simulink model "heatdrive_ecc_coupled_se21"  (R2025b)
settings: Solver=ode23t  StartTime=0.0  StopTime=10  FixedStep=0.1  MaxStep=0.4  RelTol=1e-2  AbsTol=1e-3
values from neighbouring files (symbols this model uses):
  cold_load_heat_W = 0.0    (= 0)    [Build_Simulink_Exchange_Params.m]
  cold_load_T_init = get_stage_field(stage_config, 'cold_load_T_in', get_stage_field(stage_config,          'chip_T_in', get_option_field(exchange_options, 'cold_load_T_init', get_option_field(exchange_options, 'chip_T_init', 293.0))))    [Build_Simulink_Exchange_Params.m]    (also in Create_Simulink_Exchange_Runtime.m = get_option_field(options, 'cold_load_T_init',          get_o)
  cold_sink_T_init = get_stage_field(stage_config, 'cold_sink_T_in', get_option_field(exchange_options, 'cold_sink_T_init', 293.0))    [Build_Simulink_Exchange_Params.m]    (also in Create_Simulink_Exchange_Runtime.m = get_option_field(options, 'cold_sink_T_init', ambient_T_init)
  hot_sink_T_init = get_stage_field(stage_config, 'hot_sink_T_in', get_option_field(exchange_options, 'hot_sink_T_init', 293.0))    [Build_Simulink_Exchange_Params.m]    (also in Create_Simulink_Exchange_Runtime.m = get_option_field(options, 'hot_sink_T_init', ambient_T_init))
  mdot_cooldown_source_kgps = mdot_target_kgps    [Build_Simulink_Exchange_Params.m]
  mdot_hold_source_kgps = mdot_target_kgps    [Build_Simulink_Exchange_Params.m]
  pressure_pi_bias_MPa = pressure_pi_dp_guess_MPa    [Build_Simulink_Exchange_Params.m]
  pressure_pi_error_filter_tau_s = max(get_option_field(exchange_options, 'pressure_pi_error_filter_tau_s', 0.002), 1.0e-5)    [Build_Simulink_Exchange_Params.m]
  pressure_pi_error_normalization_gain_kgps_inv = 1.0    (= 1)    [Build_Simulink_Exchange_Params.m]
  pressure_pi_max_MPa = pressure_pi_dp_guess_MPa + pressure_pi_margin_MPa    [Build_Simulink_Exchange_Params.m]
  shex_sink_T_init = get_option_field(exchange_options, 'shex_sink_T_init', hot_sink_T_init)    [Build_Simulink_Exchange_Params.m]
undefined symbols (not defined in the file or in its folder): constitutive_sample_time_s, constitutive_state21_initial, se_constitutive_T21_initial, se_pressure_integrator_max_MPa, se_pressure_pi_ki_MPa_per_kgps_s, se_pressure_pi_kp_MPa_per_kgps, se_pressure_pi_min_MPa, se_solver_T_init_21_internal, se_stage2_pressure_integrator_min_MPa, se_stage4_pressure_integrator_min_MPa, sma_constitutive_T21_initial, sma_mdot_stage1_source_kgps, sma_mdot_stage3_source_kgps, sma_pressure_integrator_max_MPa, sma_pressure_integrator_min_MPa, sma_pressure_pi_ki_MPa_per_kgps_s, sma_pressure_pi_kp_MPa_per_kgps, sma_pressure_pi_min_MPa, sma_solver_T_init_21_internal
libraries: fl_lib x484, nesl_utility x232, SimscapeFluids_lib x20
(part 8 of 8)

== matlab function heatdrive_ecc_coupled_se21/MATLAB Function ==
  data: v1_cold_inlet input; y output; v2_hot_return input; v3_sma_to_hot input; v4_hot_inlet input; v5_cold_return input; v6_sma_to_chip_cold input
function y = fcn(v1_cold_inlet,v2_hot_return,v3_sma_to_hot,v4_hot_inlet,v5_cold_return,v6_sma_to_chip_cold)
%#codegen
y = [v1_cold_inlet, v2_hot_return, v3_sma_to_hot, v4_hot_inlet, v5_cold_return, v6_sma_to_chip_cold];
